simulink model "TranscriticalCO2Cycle"  (R2023b)
settings: Solver=VariableStepAuto  StartTime=0.0  StopTime=10.0  RelTol=1e-3  AbsTol=1e-3
undefined symbols (not defined in the file or in its folder): CO2PropertyTables
libraries: fl_lib x29, SimscapeFluids_lib x7, nesl_utility x1
settings Model: Creator=smemusha  LastModifiedBy=smemusha
settings SolverCC: AutoScaleAbsTol=off  AlgebraicLoopSolver=TrustRegion  MaxZcPerStep=1
settings OptimizationCC: ReuseModelBlockBuffer=off
settings DebuggingCC: UnconnectedInputMsg=warning  UnconnectedOutputMsg=warning  UnconnectedLineMsg=warning  SymbolicDimsDataTypeCodeGenerationDiagnostic=none
settings ModelReferenceCC: EnableRefExpFcnMdlSchedulingChecks=on
settings SFSimCC: CustomCodeUndefinedFunction=UseInterfaceOnly
settings RTWCC: DLArmComputeVersion=19.05
settings SimscapeCC: SimscapeLogType=all  SimscapeLogSimulationStatistics=on  SimscapeLogDataHistory=10000

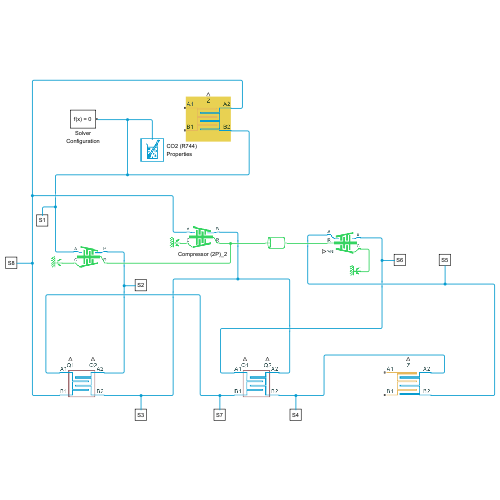
[thumbnail: Simulink's stored preview of the top-level diagram]
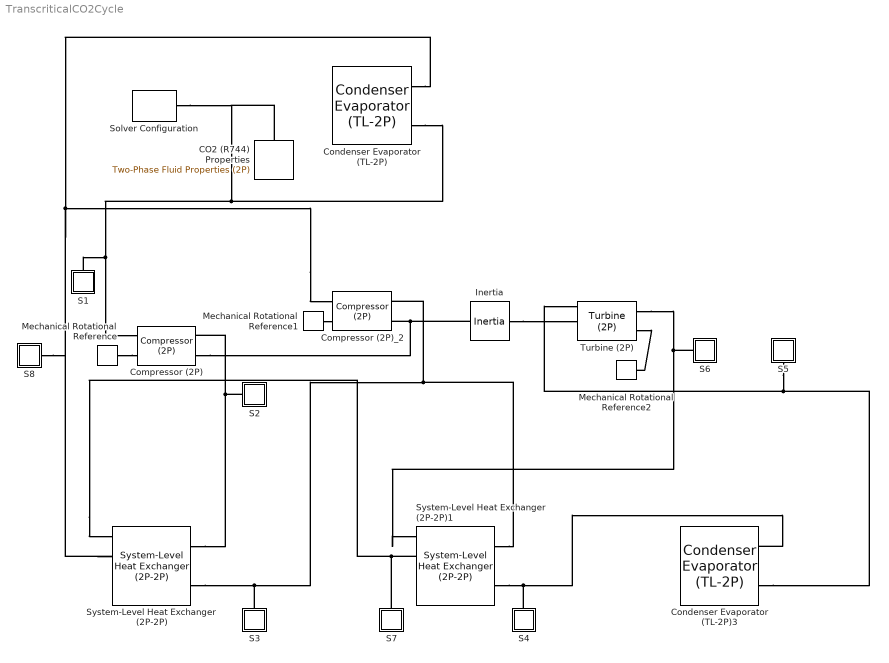
== system TranscriticalCO2Cycle ==
  CO2 (R744) Properties : fl_lib/Two-Phase Fluid/Utilities/Two-Phase Fluid Properties (2P)  u_min=CO2PropertyTables.u_min kJ/kg  u_max=CO2PropertyTables.u_max kJ/kg  p_TLU=CO2PropertyTables.p MPa  p_crit=CO2PropertyTables.p_crit MPa  critical_region=foundation.enum.critical_region.clip  p_crit_fraction=0.12  p_atm=CO2PropertyTables.p(1) MPa  properties_range_check=simscape.enum.assert.action.error  q_rev=0.01 Pa  unorm_liq=CO2PropertyTables.liquid.unorm  v_liq=CO2PropertyTables.liquid.v m^3/kg  s_liq=CO2PropertyTables.liquid.s kJ/kg/K  T_liq=CO2PropertyTables.liquid.T K  nu_liq=CO2PropertyTables.liquid.nu mm^2/s  k_liq=CO2PropertyTables.liquid.k W/(m*K)  Pr_liq=CO2PropertyTables.liquid.Pr  u_sat_liq=CO2PropertyTables.liquid.u_sat kJ/kg  unorm_vap=CO2PropertyTables.vapor.unorm  v_vap=CO2PropertyTables.vapor.v m^3/kg  s_vap=CO2PropertyTables.vapor.s kJ/kg/K  T_vap=CO2PropertyTables.vapor.T K  nu_vap=CO2PropertyTables.vapor.nu m^2/s  k_vap=CO2PropertyTables.vapor.k W/(m*K)  Pr_vap=CO2PropertyTables.vapor.Pr  u_sat_vap=CO2PropertyTables.vapor.u_sat kJ/kg
      settings: InternalSimscapePortConfiguration="{\"Bottom\":[],\"Left\":[],\"Right\":[{\"id\":\"A\",\"label\":\"\",\"type\":\"foundation.two_phase_fluid.two_phase_fluid\"}],\"Top\":[]}"
  Compressor (2P) : SimscapeFluids_lib/Two-Phase Fluid/Fluid Machines/Compressor (2P)  parameterization=fluids.two_phase_fluid.fluid_machines.enum.CompressorParameterization.Analytical  NDes=25000 rpm  piDes=2.2  mdotDes=3 kg/s  efficiencyType=fluids.two_phase_fluid.fluid_machines.enum.EfficiencyType.Analytical  efficiencyValue=0.8  etaMax=0.88  etaMin=0.8  mdotMaxEff=3.5 kg/s  piMaxEff=2.67  omega_TLU=250 .* [50, 71, 87, 100] rpm  beta_TLU=0 : 1 / 5 : 1  pr_TLU=[1.1814, 1.2385, 1.2792, 1.3017, 1.3057, 1.3057; 1.3648, 1.5157, 1.6298, 1.691, 1.7011, 1.7032; 1.587, 1.8357, 2.011, 2.0925, 2.1006, 2.1006; 1.8255, 2.28, 2.4777, 2.5225, 2.5633, 2.5389]  mdot_TLU=[.1503, .1313, .11, .0887, .0668, .0502; .2265, .1999, .1649, .1322, .0992, .0639; .2869, .2545, .216, .1798, .1424, .108; .3275, .2846, .2466, .2285, .209, .1661] kg/s  eta_TLU=[.56, .66, .71, .695, .659, .635; .558, .682, .755, .743, .697, .638; .57, .705, .765, .752, .712, .652; .552, .718, .755, .752, .736, .67]  SMFault=simscape.enum.assert.action.none  a=1.5  b=5  k=0.03  c=3  d=4  cCap=15  dCap=1.0  p_reference=0.101325 MPa  T_reference=373.15 K  mechanical_efficiency=0.9  area_A=0.01 m^2  area_B=0.01 m^2  VaporCheck=simscape.enum.assert.action.warn
      settings: InternalSimscapePortConfiguration="{\"Bottom\":[],\"Left\":[{\"id\":\"A\",\"label\":\"A\",\"type\":\"foundation.two_phase_fluid.two_phase_fluid\"},{\"id\":\"C\",\"label\":\"C\",\"type\":\"foundation.mechanical.rotational.rotational\"}],\"Right\":[{\"id\":\"B\",\"label\":\"B\",\"type\":\"foundation.two_phase_fluid.two_phase_fluid\"},{\"id\":\"R\",\"label\":\"R\",\"type\":\"foundation.mechanical.rotational.rotational\"}],\"Top\":[]}"
  Compressor (2P)_2 : SimscapeFluids_lib/Two-Phase Fluid/Fluid Machines/Compressor (2P)  parameterization=fluids.two_phase_fluid.fluid_machines.enum.CompressorParameterization.Analytical  NDes=25000 rpm  piDes=2.2  mdotDes=0.20 kg/s  efficiencyType=fluids.two_phase_fluid.fluid_machines.enum.EfficiencyType.Analytical  efficiencyValue=0.8  etaMax=0.887  etaMin=0.5  mdotMaxEff=0.19 kg/s  piMaxEff=2.1  omega_TLU=250 .* [50, 71, 87, 100] rpm  beta_TLU=0 : 1 / 5 : 1  pr_TLU=[1.1814, 1.2385, 1.2792, 1.3017, 1.3057, 1.3057; 1.3648, 1.5157, 1.6298, 1.691, 1.7011, 1.7032; 1.587, 1.8357, 2.011, 2.0925, 2.1006, 2.1006; 1.8255, 2.28, 2.4777, 2.5225, 2.5633, 2.5389]  mdot_TLU=[.1503, .1313, .11, .0887, .0668, .0502; .2265, .1999, .1649, .1322, .0992, .0639; .2869, .2545, .216, .1798, .1424, .108; .3275, .2846, .2466, .2285, .209, .1661] kg/s  eta_TLU=[.56, .66, .71, .695, .659, .635; .558, .682, .755, .743, .697, .638; .57, .705, .765, .752, .712, .652; .552, .718, .755, .752, .736, .67]  SMFault=simscape.enum.assert.action.none  a=1.5  b=5  k=0.03  c=3  d=4  cCap=15  dCap=1.0  p_reference=0.101325 MPa  T_reference=373.15 K  mechanical_efficiency=0.9  area_A=0.01 m^2  area_B=0.01 m^2  VaporCheck=simscape.enum.assert.action.warn
      settings: InternalSimscapePortConfiguration="{\"Bottom\":[],\"Left\":[{\"id\":\"A\",\"label\":\"A\",\"type\":\"foundation.two_phase_fluid.two_phase_fluid\"},{\"id\":\"C\",\"label\":\"C\",\"type\":\"foundation.mechanical.rotational.rotational\"}],\"Right\":[{\"id\":\"B\",\"label\":\"B\",\"type\":\"foundation.two_phase_fluid.two_phase_fluid\"},{\"id\":\"R\",\"label\":\"R\",\"type\":\"foundation.mechanical.rotational.rotational\"}],\"Top\":[]}"
  Condenser Evaporator (TL-2P) : SimscapeFluids_lib/Fluid Network Interfaces/Heat Exchangers/Condenser Evaporator (TL-2P)  flow_arrangement=fluids.interfaces.heat_exchangers.enum.FlowArrangementTL2P.Cross  cross_flow_arrangement=fluids.interfaces.heat_exchangers.enum.CrossFlowArrangementTL2P.UnmixedUnmixed  R_wall=0 K/kW  area_A1=0.01 m^2  area_B1=0.01 m^2  area_A2=0.01 m^2  area_B2=0.01 m^2  flow_geometry_TL=fluids.interfaces.heat_exchangers.enum.FlowGeometryTL.InsideTubes  tube_num_TL=25  tube_length_TL=1 m  tube_cross_section_TL=fluids.interfaces.heat_exchangers.enum.TubeCrossSection.Circular  tube_diameter_TL=0.05 m  tube_width_TL=0.05 m  tube_height_TL=0.05 m  tube_inner_diameter_TL=0.05 m  tube_outer_diameter_TL=0.1 m  tube_flow_area_TL=0.002 m^2  tube_wetted_perimeter_TL=0.15 m  tube_heat_perimeter_TL=0.15 m  tube_pressure_loss_spec_TL=fluids.interfaces.heat_exchangers.enum.TubePressureLossSpec.Haaland  tube_loss_coeff_TL=10  tube_local_pressure_loss_spec_TL=fluids.thermal_liquid.pipes_fittings.enum.LocalLossSpec.AggregateLength  tube_length_add_TL=0.1 m  tube_local_loss_coefficient_TL=0.1  tube_roughness_pressure_TL=15e-6 m  tube_Re_lam_pressure_TL=2000  tube_Re_tur_pressure_TL=4000  tube_shape_factor_generic_TL=64  tube_heat_coeff_spec_TL=fluids.interfaces.heat_exchangers.enum.TubeHeatCoeffSpec.Gneilinski  tube_colburn_coeff_TL=[.023, .8, .33]  tube_roughness_heat_TL=15e-6 m  tube_Re_lam_heat_TL=2000  tube_Re_tur_heat_TL=4000  tube_Nu_lam_generic_TL=3.66  bank_arrangement_TL=fluids.interfaces.heat_exchangers.enum.BankArrangement.Inline  bank_num_rows_TL=5  bank_tubes_per_row_TL=5  bank_width_TL=1 m  bank_tube_diameter_TL=0.05 m  bank_longitudinal_pitch_TL=0.15 m  bank_transverse_pitch_TL=0.15 m  bank_pressure_loss_spec_TL=fluids.interfaces.heat_exchangers.enum.BankPressureLossSpec.Martin  bank_euler_TL=10  bank_heat_coeff_spec_TL=fluids.interfaces.heat_exchangers.enum.BankHeatCoeffSpec.Martin  bank_colburn_coeff_TL=[.27, .63, .36]  generic_flow_area_TL=0.01 m^2  generic_heat_area_TL=2 m^2  generic_volume_TL=0.05 m^3  generic_loss_coeff_TL=10  generic_colburn_coeff_TL=[.023, .8, .33]  fouling_factor_TL=0.1 K*m^2/kW  fin_area_TL=0 m^2  fin_efficiency_TL=0.5  p_init_TL=7.5 MPa  T_init_TL=305 K  tube_num_2P=25  tube_length_2P=1 m  tube_cross_section_2P=fluids.interfaces.heat_exchangers.enum.TubeCrossSection.Circular  tube_diameter_2P=0.05 m  tube_width_2P=0.05 m  tube_height_2P=0.05 m  tube_inner_diameter_2P=0.05 m  tube_outer_diameter_2P=0.1 m  tube_flow_area_2P=0.002 m^2  tube_wetted_perimeter_2P=0.15 m  tube_heat_perimeter_2P=0.15 m  tube_pressure_loss_spec_2P=fluids.interfaces.heat_exchangers.enum.TubePressureLossSpec2P.Haaland  tube_loss_coeff_2P=10  tube_local_pressure_loss_spec_2P=fluids.two_phase_fluid.pipes_fittings.enum.LocalLossSpec.AggregateLength  tube_length_add_2P=0.1 m  tube_local_loss_coefficient_2P=0.1  tube_roughness_pressure_2P=15e-6 m  tube_Re_lam_pressure_2P=2000  tube_Re_tur_pressure_2P=4000  tube_shape_factor_generic_2P=64  tube_heat_coeff_spec_2P=fluids.interfaces.heat_exchangers.enum.TubeHeatCoeffSpec2P.GneilinskiCavalliniZecchin  tube_colburn_coeff_liq_2P=[.023, .8, .33]  tube_colburn_coeff_mix_2P=[.05, .8, .33]  tube_colburn_coeff_vap_2P=[.023, .8, .33]  tube_roughness_heat_2P=15e-6 m  tube_Re_lam_heat_2P=2000  tube_Re_tur_heat_2P=4000  tube_Nu_lam_generic_2P=3.66  fouling_factor_2P=0.1 K*m^2/kW  fin_area_2P=0 m^2  fin_efficiency_2P=0.5  energy_spec_2P=foundation.enum.energy_spec.temperature  p_init_2P=0.101325 MPa  T_init_2P=293.15 K  x_init_2P=0.5  alpha_init_2P=0.5  h_init_2P=1500 kJ/kg  u_init_2P=1500 kJ/kg
      settings: InternalSimscapePortConfiguration="{\"Bottom\":[],\"Left\":[{\"id\":\"A1\",\"label\":\"A1\",\"type\":\"foundation.thermal_liquid.thermal_liquid\"},{\"id\":\"B1\",\"label\":\"B1\",\"type\":\"foundation.thermal_liquid.thermal_liquid\"}],\"Right\":[{\"id\":\"A2\",\"label\":\"A2\",\"type\":\"foundation.two_phase_fluid.two_phase_fluid\"},{\"id\":\"B2\",\"label\":\"B2\",\"type\":\"foundation.two_phase_fluid.two_phase_fluid\"}],\"Top\":[{\"id\":\"Z\",\"label\":\"Z\",\"type\":\"output\"}]}"
  Condenser Evaporator (TL-2P)3 : SimscapeFluids_lib/Fluid Network Interfaces/Heat Exchangers/Condenser Evaporator (TL-2P)  flow_arrangement=fluids.interfaces.heat_exchangers.enum.FlowArrangementTL2P.Cross  cross_flow_arrangement=fluids.interfaces.heat_exchangers.enum.CrossFlowArrangementTL2P.UnmixedUnmixed  R_wall=0 K/kW  area_A1=0.01 m^2  area_B1=0.01 m^2  area_A2=0.01 m^2  area_B2=0.01 m^2  flow_geometry_TL=fluids.interfaces.heat_exchangers.enum.FlowGeometryTL.InsideTubes  tube_num_TL=25  tube_length_TL=1 m  tube_cross_section_TL=fluids.interfaces.heat_exchangers.enum.TubeCrossSection.Circular  tube_diameter_TL=0.05 m  tube_width_TL=0.05 m  tube_height_TL=0.05 m  tube_inner_diameter_TL=0.05 m  tube_outer_diameter_TL=0.1 m  tube_flow_area_TL=0.002 m^2  tube_wetted_perimeter_TL=0.15 m  tube_heat_perimeter_TL=0.15 m  tube_pressure_loss_spec_TL=fluids.interfaces.heat_exchangers.enum.TubePressureLossSpec.Haaland  tube_loss_coeff_TL=10  tube_local_pressure_loss_spec_TL=fluids.thermal_liquid.pipes_fittings.enum.LocalLossSpec.AggregateLength  tube_length_add_TL=0.1 m  tube_local_loss_coefficient_TL=0.1  tube_roughness_pressure_TL=15e-6 m  tube_Re_lam_pressure_TL=2000  tube_Re_tur_pressure_TL=4000  tube_shape_factor_generic_TL=64  tube_heat_coeff_spec_TL=fluids.interfaces.heat_exchangers.enum.TubeHeatCoeffSpec.Gneilinski  tube_colburn_coeff_TL=[.023, .8, .33]  tube_roughness_heat_TL=15e-6 m  tube_Re_lam_heat_TL=2000  tube_Re_tur_heat_TL=4000  tube_Nu_lam_generic_TL=3.66  bank_arrangement_TL=fluids.interfaces.heat_exchangers.enum.BankArrangement.Inline  bank_num_rows_TL=5  bank_tubes_per_row_TL=5  bank_width_TL=1 m  bank_tube_diameter_TL=0.05 m  bank_longitudinal_pitch_TL=0.15 m  bank_transverse_pitch_TL=0.15 m  bank_pressure_loss_spec_TL=fluids.interfaces.heat_exchangers.enum.BankPressureLossSpec.Martin  bank_euler_TL=10  bank_heat_coeff_spec_TL=fluids.interfaces.heat_exchangers.enum.BankHeatCoeffSpec.Martin  bank_colburn_coeff_TL=[.27, .63, .36]  generic_flow_area_TL=0.01 m^2  generic_heat_area_TL=2 m^2  generic_volume_TL=0.05 m^3  generic_loss_coeff_TL=10  generic_colburn_coeff_TL=[.023, .8, .33]  fouling_factor_TL=0.1 K*m^2/kW  fin_area_TL=0 m^2  fin_efficiency_TL=0.5  p_init_TL=0.101325 MPa  T_init_TL=293.15 K  tube_num_2P=25  tube_length_2P=1 m  tube_cross_section_2P=fluids.interfaces.heat_exchangers.enum.TubeCrossSection.Circular  tube_diameter_2P=0.05 m  tube_width_2P=0.05 m  tube_height_2P=0.05 m  tube_inner_diameter_2P=0.05 m  tube_outer_diameter_2P=0.1 m  tube_flow_area_2P=0.002 m^2  tube_wetted_perimeter_2P=0.15 m  tube_heat_perimeter_2P=0.15 m  tube_pressure_loss_spec_2P=fluids.interfaces.heat_exchangers.enum.TubePressureLossSpec2P.Haaland  tube_loss_coeff_2P=10  tube_local_pressure_loss_spec_2P=fluids.two_phase_fluid.pipes_fittings.enum.LocalLossSpec.AggregateLength  tube_length_add_2P=0.1 m  tube_local_loss_coefficient_2P=0.1  tube_roughness_pressure_2P=15e-6 m  tube_Re_lam_pressure_2P=2000  tube_Re_tur_pressure_2P=4000  tube_shape_factor_generic_2P=64  tube_heat_coeff_spec_2P=fluids.interfaces.heat_exchangers.enum.TubeHeatCoeffSpec2P.GneilinskiCavalliniZecchin  tube_colburn_coeff_liq_2P=[.023, .8, .33]  tube_colburn_coeff_mix_2P=[.05, .8, .33]  tube_colburn_coeff_vap_2P=[.023, .8, .33]  tube_roughness_heat_2P=15e-6 m  tube_Re_lam_heat_2P=2000  tube_Re_tur_heat_2P=4000  tube_Nu_lam_generic_2P=3.66  fouling_factor_2P=0.1 K*m^2/kW  fin_area_2P=0 m^2  fin_efficiency_2P=0.5  energy_spec_2P=foundation.enum.energy_spec.temperature  p_init_2P=0.101325 MPa  T_init_2P=293.15 K  x_init_2P=0.5  alpha_init_2P=0.5  h_init_2P=1500 kJ/kg  u_init_2P=1500 kJ/kg
      settings: InternalSimscapePortConfiguration="{\"Bottom\":[],\"Left\":[{\"id\":\"A1\",\"label\":\"A1\",\"type\":\"foundation.thermal_liquid.thermal_liquid\"},{\"id\":\"B1\",\"label\":\"B1\",\"type\":\"foundation.thermal_liquid.thermal_liquid\"}],\"Right\":[{\"id\":\"A2\",\"label\":\"A2\",\"type\":\"foundation.two_phase_fluid.two_phase_fluid\"},{\"id\":\"B2\",\"label\":\"B2\",\"type\":\"foundation.two_phase_fluid.two_phase_fluid\"}],\"Top\":[{\"id\":\"Z\",\"label\":\"Z\",\"type\":\"output\"}]}"
  Inertia : fl_lib/Mechanical/Rotational Elements/Inertia  inertia=shaft_inertia kg*m^2  num_ports=foundation.enum.numPorts2.two  w_specify=on  w_priority=High  w=10000 rpm  w_nominal_specify=off  w_nominal_unit=rad/s  w_nominal_value=1  t_specify=off  t_priority=None  t=0 N*m  t_nominal_specify=off  t_nominal_unit=N*m  t_nominal_value=1
      settings: InternalSimscapePortConfiguration="{\"Bottom\":[],\"Left\":[{\"id\":\"I\",\"label\":\"\",\"type\":\"foundation.mechanical.rotational.rotational\"}],\"Right\":[{\"id\":\"J\",\"label\":\"\",\"type\":\"foundation.mechanical.rotational.rotational\"}],\"Top\":[]}"
  Mechanical Rotational Reference : fl_lib/Mechanical/Rotational Elements/Mechanical Rotational Reference
  Mechanical Rotational Reference1 : fl_lib/Mechanical/Rotational Elements/Mechanical Rotational Reference
  Mechanical Rotational Reference2 : fl_lib/Mechanical/Rotational Elements/Mechanical Rotational Reference
  S1 : Subsystem
      mask Display: disp(get_param(gcb, 'Name'))
  S2 : Subsystem
      settings: PortSchema="{\"entries\":[{\"content\":{\"sides\":[{\"content\":{},\"type\":\"ConnectorPlacement.EquallySpacedRectSide\",\"uuid\":\"af0e4199-d47a-4ec0-94eb-7962f8049a35\"},{\"content\":{\"side\":\"RIGHT\"},\"type\":\"ConnectorPlacement.EquallySpacedRectSide\",\"uuid\":\"e53baceb-841d-4d18-830d-da2777b33e2d\"},{\"content\":{\"connectorIds\":[\"LConn1\"],\"side\":\"TOP\"},\"type\":\"ConnectorPlacement.EquallySpacedRectSide\",\"uuid\":\"c9dd45b9-7dec-4baa-8c3e-b872dab8c4af\"}]},\"type\":\"ConnectorPlacement.EquallySpacedConnector\",\"uuid\":\"6eb31624-81b7-422d-8922-37e9cf91a1f7\"}],\"packageUris\":[\"http://schema.mathworks.com/mf0/Connector/R2020b\"],\"version\":\"1.0\"}"
      mask Display: disp(get_param(gcb, 'Name'))
  S3 : Subsystem
      mask Display: disp(get_param(gcb, 'Name'))
  S4 : Subsystem
      mask Display: disp(get_param(gcb, 'Name'))
  S5 : Subsystem
      mask Display: disp(get_param(gcb, 'Name'))
  S6 : Subsystem
      settings: PortSchema="{\"entries\":[{\"content\":{\"sides\":[{\"content\":{},\"type\":\"ConnectorPlacement.EquallySpacedRectSide\",\"uuid\":\"af0e4199-d47a-4ec0-94eb-7962f8049a35\"},{\"content\":{\"side\":\"RIGHT\"},\"type\":\"ConnectorPlacement.EquallySpacedRectSide\",\"uuid\":\"e53baceb-841d-4d18-830d-da2777b33e2d\"},{\"content\":{\"connectorIds\":[\"LConn1\"],\"side\":\"TOP\"},\"type\":\"ConnectorPlacement.EquallySpacedRectSide\",\"uuid\":\"c9dd45b9-7dec-4baa-8c3e-b872dab8c4af\"}]},\"type\":\"ConnectorPlacement.EquallySpacedConnector\",\"uuid\":\"6eb31624-81b7-422d-8922-37e9cf91a1f7\"}],\"packageUris\":[\"http://schema.mathworks.com/mf0/Connector/R2020b\"],\"version\":\"1.0\"}"
      mask Display: disp(get_param(gcb, 'Name'))
  S7 : Subsystem
      mask Display: disp(get_param(gcb, 'Name'))
  S8 : Subsystem
      settings: PortSchema="{\"entries\":[{\"content\":{\"sides\":[{\"content\":{},\"type\":\"ConnectorPlacement.EquallySpacedRectSide\",\"uuid\":\"af0e4199-d47a-4ec0-94eb-7962f8049a35\"},{\"content\":{\"side\":\"RIGHT\"},\"type\":\"ConnectorPlacement.EquallySpacedRectSide\",\"uuid\":\"e53baceb-841d-4d18-830d-da2777b33e2d\"},{\"content\":{\"side\":\"TOP\"},\"type\":\"ConnectorPlacement.EquallySpacedRectSide\",\"uuid\":\"c9dd45b9-7dec-4baa-8c3e-b872dab8c4af\"},{\"content\":{\"connectorIds\":[\"RConn1\"],\"side\":\"BOTTOM\"},\"type\":\"ConnectorPlacement.EquallySpacedRectSide\",\"uuid\":\"10f1a485-95f0-4282-b277-18e46c743bab\"}]},\"type\":\"ConnectorPlacement.EquallySpacedConnector\",\"uuid\":\"6eb31624-81b7-422d-8922-37e9cf91a1f7\"}],\"packageUris\":[\"http://schema.mathworks.com/mf0/Connector/R2020b\"],\"version\":\"1.0\"}"
      mask Display: disp(get_param(gcb, 'Name'))
  Solver Configuration : nesl_utility/Solver Configuration  PhysicalDomain=network_engine_domain  SubClassName=solver  LeftPortType=input  RightPortType=generic  Tones=[]  Harmonics=[]  SimulateNoise=off  Profile=off  UseLocalSampling=off  EnableSwitchedLinearOptims=on  FrequencyDomain=off  UseCCode=off  RelTol=0.001  AbsTol=1e-06  MinStep=1e-09  ToWorkspace=off  RevertToSquareIcSolve=off  NumHomotopyIterations=100  PhasorMode=off  PhasorModeNumHarmonics=1  ConsistencySolver=NEWTON_XTOL_AFTER_FTOL  IndexReductionMethod=DerivativeReplacement  DoDC=off  ResidualTolerance=1e-09  ConsistencyTolSource=GLOBAL  ConsistencyAbsTol=0.001  ConsistencyRelTol=0.001  ConsistencyTolFactor=0.001  UseLocalSolver=off  LocalSolverChoice=NE_BACKWARD_EULER_ADVANCER  ResolveIndetEquations=on  FunctionEvalNumThread=1  LocalSolverSampleTime=0.001  DoFixedCost=off  MaxNonlinIter=3  MaxModeIter=2  ComputeImpulses=off  ImpulseIterations=2  LinearAlgebra=auto  LinearAlgebraNumThread=0  EquationFormulation=NE_TIME_EF  DelaysMemoryBudget=1024  AutomaticFiltering=on  FilteringTimeConstant=0.001  PartitionStorageMethod=AS_NEEDED  PartitionMemoryBudget=1024  PartitionMethod=ROBUST  MultibodyUseLocalSolver=off  MultibodyLocalSolverChoice=ODE1  MultibodyLocalSolverSampleTime=0.001
  System-Level Heat Exchanger (2P-2P) : SimscapeFluids_lib/Fluid Network Interfaces/Heat Exchangers/System-Level Heat Exchanger (2P-2P)  flow_arrangement=fluids.interfaces.heat_exchangers.enum.SystemLevelFlowArrangement2P2P.Counter  wall_thermal_mass=false  mass_wall=1 kg  cp_wall=490 J/(K*kg)  nominal_init_wall=true  T_wall_init=293.15 K  area_A1=0.01 m^2  area_B1=0.01 m^2  area_A2=0.01 m^2  area_B2=0.01 m^2  operating_condition_2P1=fluids.interfaces.heat_exchangers.enum.SystemLevelOperatingCondition2P2P.Cooling  mdot_nominal_2P1=0.001 kg/s  delta_p_nominal_2P1=0.01 MPa  pressure_spec_2P1=fluids.interfaces.heat_exchangers.enum.SystemLevelPressureSpec2P.InletPressure  p_in_nominal_2P1=1 MPa  T_sat_nominal_2P1=313.15 K  inlet_spec_2P1=fluids.interfaces.heat_exchangers.enum.SystemLevelInletSpec2P.Enthalpy  T_in_nominal_2P1=333.15 K  h_in_nominal_2P1=440 kJ/kg  x_in_nominal_2P1=1  capacity_spec_2P1=fluids.interfaces.heat_exchangers.enum.SystemLevelCapacitySpec.HeatTransfer  Q_nominal=0.1 kW  outlet_spec_cool_2P1=fluids.interfaces.heat_exchangers.enum.SystemLevelOutletSpecCondenser2P.Enthalpy  outlet_spec_heat_2P1=fluids.interfaces.heat_exchangers.enum.SystemLevelOutletSpecEvaporator2P.Enthalpy  delta_T_sub_nominal_2P1=5 deltaK  delta_T_sup_nominal_2P1=5 deltaK  h_out_nominal_2P1=250 kJ/kg  x_out_nominal_2P1=0  volume_2P1=0.001 m^3  nominal_init_2P1=true  energy_spec_2P1=foundation.enum.energy_spec.enthalpy  p_init_2P1=0.101325 MPa  T_init_2P1=293.15 K  x_init_2P1=0.5  alpha_init_2P1=0.5  h_init_2P1=1500 kJ/kg  u_init_2P1=1500 kJ/kg  mdot_nominal_2P2=0.001 kg/s  delta_p_nominal_2P2=0.01 MPa  pressure_spec_2P2=fluids.interfaces.heat_exchangers.enum.SystemLevelPressureSpec2P.InletPressure  p_in_nominal_2P2=0.1 MPa  T_sat_nominal_2P2=243.15 K  inlet_spec_2P2=fluids.interfaces.heat_exchangers.enum.SystemLevelInletSpec2P.Enthalpy  T_in_nominal_2P2=237.15 K  h_in_nominal_2P2=230 kJ/kg  x_in_nominal_2P2=0.1  volume_2P2=0.001 m^3  nominal_init_2P2=true  energy_spec_2P2=foundation.enum.energy_spec.enthalpy  p_init_2P2=0.101325 MPa  T_init_2P2=293.15 K  x_init_2P2=0.5  alpha_init_2P2=0.5  h_init_2P2=1500 kJ/kg  u_init_2P2=1500 kJ/kg  a_liq_2P1=0.023  a_mix_2P1=0.005  a_vap_2P1=0.023  b_2P1=0.8  c_2P1=0.33  a_liq_2P2=0.023  a_mix_2P2=0.005  a_vap_2P2=0.023  b_2P2=0.8  c_2P2=0.33
      settings: InternalSimscapePortConfiguration="{\"Bottom\":[],\"Left\":[{\"id\":\"A1\",\"label\":\"A1\",\"type\":\"foundation.two_phase_fluid.two_phase_fluid\"},{\"id\":\"B1\",\"label\":\"B1\",\"type\":\"foundation.two_phase_fluid.two_phase_fluid\"}],\"Right\":[{\"id\":\"A2\",\"label\":\"A2\",\"type\":\"foundation.two_phase_fluid.two_phase_fluid\"},{\"id\":\"B2\",\"label\":\"B2\",\"type\":\"foundation.two_phase_fluid.two_phase_fluid\"}],\"Top\":[{\"id\":\"Q1\",\"label\":\"Q1\",\"type\":\"output\"},{\"id\":\"Q2\",\"label\":\"Q2\",\"type\":\"output\"}]}"
  System-Level Heat Exchanger (2P-2P)1 : SimscapeFluids_lib/Fluid Network Interfaces/Heat Exchangers/System-Level Heat Exchanger (2P-2P)  flow_arrangement=fluids.interfaces.heat_exchangers.enum.SystemLevelFlowArrangement2P2P.Counter  wall_thermal_mass=false  mass_wall=1 kg  cp_wall=490 J/(K*kg)  nominal_init_wall=true  T_wall_init=293.15 K  area_A1=0.01 m^2  area_B1=0.01 m^2  area_A2=0.01 m^2  area_B2=0.01 m^2  operating_condition_2P1=fluids.interfaces.heat_exchangers.enum.SystemLevelOperatingCondition2P2P.Cooling  mdot_nominal_2P1=0.001 kg/s  delta_p_nominal_2P1=0.01 MPa  pressure_spec_2P1=fluids.interfaces.heat_exchangers.enum.SystemLevelPressureSpec2P.InletPressure  p_in_nominal_2P1=1 MPa  T_sat_nominal_2P1=313.15 K  inlet_spec_2P1=fluids.interfaces.heat_exchangers.enum.SystemLevelInletSpec2P.Enthalpy  T_in_nominal_2P1=333.15 K  h_in_nominal_2P1=440 kJ/kg  x_in_nominal_2P1=1  capacity_spec_2P1=fluids.interfaces.heat_exchangers.enum.SystemLevelCapacitySpec.HeatTransfer  Q_nominal=0.1 kW  outlet_spec_cool_2P1=fluids.interfaces.heat_exchangers.enum.SystemLevelOutletSpecCondenser2P.Enthalpy  outlet_spec_heat_2P1=fluids.interfaces.heat_exchangers.enum.SystemLevelOutletSpecEvaporator2P.Enthalpy  delta_T_sub_nominal_2P1=5 deltaK  delta_T_sup_nominal_2P1=5 deltaK  h_out_nominal_2P1=250 kJ/kg  x_out_nominal_2P1=0  volume_2P1=0.001 m^3  nominal_init_2P1=true  energy_spec_2P1=foundation.enum.energy_spec.enthalpy  p_init_2P1=0.101325 MPa  T_init_2P1=293.15 K  x_init_2P1=0.5  alpha_init_2P1=0.5  h_init_2P1=1500 kJ/kg  u_init_2P1=1500 kJ/kg  mdot_nominal_2P2=0.001 kg/s  delta_p_nominal_2P2=0.01 MPa  pressure_spec_2P2=fluids.interfaces.heat_exchangers.enum.SystemLevelPressureSpec2P.InletPressure  p_in_nominal_2P2=0.1 MPa  T_sat_nominal_2P2=243.15 K  inlet_spec_2P2=fluids.interfaces.heat_exchangers.enum.SystemLevelInletSpec2P.Enthalpy  T_in_nominal_2P2=237.15 K  h_in_nominal_2P2=230 kJ/kg  x_in_nominal_2P2=0.1  volume_2P2=0.001 m^3  nominal_init_2P2=true  energy_spec_2P2=foundation.enum.energy_spec.enthalpy  p_init_2P2=0.101325 MPa  T_init_2P2=293.15 K  x_init_2P2=0.5  alpha_init_2P2=0.5  h_init_2P2=1500 kJ/kg  u_init_2P2=1500 kJ/kg  a_liq_2P1=0.023  a_mix_2P1=0.005  a_vap_2P1=0.023  b_2P1=0.8  c_2P1=0.33  a_liq_2P2=0.023  a_mix_2P2=0.005  a_vap_2P2=0.023  b_2P2=0.8  c_2P2=0.33
      settings: InternalSimscapePortConfiguration="{\"Bottom\":[],\"Left\":[{\"id\":\"A1\",\"label\":\"A1\",\"type\":\"foundation.two_phase_fluid.two_phase_fluid\"},{\"id\":\"B1\",\"label\":\"B1\",\"type\":\"foundation.two_phase_fluid.two_phase_fluid\"}],\"Right\":[{\"id\":\"A2\",\"label\":\"A2\",\"type\":\"foundation.two_phase_fluid.two_phase_fluid\"},{\"id\":\"B2\",\"label\":\"B2\",\"type\":\"foundation.two_phase_fluid.two_phase_fluid\"}],\"Top\":[{\"id\":\"Q1\",\"label\":\"Q1\",\"type\":\"output\"},{\"id\":\"Q2\",\"label\":\"Q2\",\"type\":\"output\"}]}"
  Turbine (2P) : SimscapeFluids_lib/Two-Phase Fluid/Fluid Machines/Turbine (2P)  parameterization=fluids.two_phase_fluid.fluid_machines.enum.TurbineParameterization.Analytical  omega_TLU_2=250 .* [50, 60, 70, 80, 90, 100, 110] rpm  variable_nozzle=true  min_nozzle_opening=1e-3  max_nozzle_opening=1  pr_nom=2.67  mdot_nom=3 kg/s  pr_mdot_TLU=[1.251, 1.345, 1.442, 1.521, 1.596, 1.692, 1.849, 1.972, 2.1, 2.173, 2.259, 2.3424]  mdot_TLU=0.01 .* [39.439, 43.01, 45.556, 46.801, 47.792, 48.388, 48.634, 48.67, 48.689, 48.747, 48.825, 48.912] kg/s  pr_mdot_TLU_2=[1.217, 1.285, 1.323, 1.363, 1.402, 1.427, 1.495, 1.545, 1.6, 1.687, 1.747, 1.8074; 1.231, 1.302, 1.356, 1.404, 1.443, 1.473, 1.525, 1.577, 1.635, 1.709, 1.782, 1.845; 1.242, 1.328, 1.388, 1.437, 1.528, 1.617, 1.704, 1.811, 1.915, 1.979, 2.053, 2.1226; 1.244, 1.339, 1.417, 1.465, 1.528, 1.584, 1.692, 1.787, 1.899, 2, 2.075, 2.1492; 1.245, 1.34, 1.425, 1.492, 1.546, 1.684, 1.748, 1.882, 1.987, 2.084, 2.167, 2.2458; 1.251, 1.345, 1.442, 1.521, 1.596, 1.692, 1.849, 1.972, 2.1, 2.173, 2.259, 2.3424; 1.248, 1.348, 1.447, 1.516, 1.581, 1.651, 1.749, 1.839, 1.93, 2.024, 2.154, 2.242]  mdot_TLU_2=0.01 .* [40.403, 44.417, 46.653, 47.966, 48.97, 49.544, 50.001, 50.081, 50.086, 50.095, 50.09, 50.0922; 40.044, 43.754, 46.125, 47.626, 48.513, 49.105, 49.481, 49.58, 49.597, 49.624, 49.638, 49.633; 39.941, 43.795, 46.017, 47.335, 48.795, 49.199, 49.279, 49.27, 49.248, 49.23, 49.255, 49.2428; 39.896, 43.512, 45.914, 47.061, 48.011, 48.558, 48.943, 49.042, 49.069, 49.01, 49.046, 49.0266; 39.524, 42.934, 45.686, 46.743, 47.715, 48.67, 48.777, 48.836, 48.876, 48.836, 48.845, 48.8184; 39.439, 43.01, 45.556, 46.801, 47.792, 48.388, 48.634, 48.67, 48.639, 48.647, 48.625, 48.5912; 39.502, 42.849, 45.336, 46.385, 47.312, 47.877, 48.222, 48.397, 48.459, 48.482, 48.455, 48.414] kg/s  efficiency_constant=0.9  pr_eta_TLU=[1.252, 1.328, 1.425, 1.544, 1.642, 1.757, 1.873, 2.005, 2.1, 2.204, 2.248, 2.28]  eta_TLU=[.559, .61, .673, .741, .788, .835, .869, .895, .908, .899, .854, .751]  pr_eta_TLU_2=[1.224, 1.246, 1.292, 1.387, 1.457, 1.534, 1.61, 1.686, 1.743, 1.79, 1.871, 1.914; 1.237, 1.25, 1.28, 1.369, 1.459, 1.553, 1.629, 1.716, 1.799, 1.846, 1.927, 1.97; 1.241, 1.255, 1.283, 1.326, 1.401, 1.509, 1.591, 1.704, 1.806, 1.913, 1.994, 2.037; 1.25, 1.265, 1.308, 1.364, 1.456, 1.532, 1.637, 1.739, 1.851, 1.934, 2.042, 2.085; 1.281, 1.314, 1.371, 1.425, 1.498, 1.574, 1.647, 1.749, 1.878, 1.979, 2.091, 2.18; 1.252, 1.328, 1.425, 1.544, 1.642, 1.757, 1.873, 2.005, 2.1, 2.204, 2.248, 2.28; 1.382, 1.43, 1.495, 1.586, 1.688, 1.791, 1.887, 1.99, 2.079, 2.158, 2.249, 2.36]  eta_TLU_2=[.72, .754, .759, .739, .714, .679, .643, .603, .554, .524, .494, .48; .716, .757, .794, .819, .812, .788, .761, .728, .692, .662, .632, .618; .629, .691, .775, .831, .858, .869, .859, .842, .816, .782, .752, .738; .594, .668, .757, .804, .857, .883, .892, .893, .884, .865, .835, .821; .664, .72, .779, .823, .858, .883, .897, .905, .904, .896, .883, .868; .559, .61, .673, .741, .788, .835, .869, .895, .908, .899, .854, .751; .718, .785, .824, .855, .882, .9, .908, .906, .884, .857, .804, .701]  p_reference=0.101325 MPa  T_reference=373.15 K  mechanical_efficiency=0.9  area_A=0.01 m^2  area_B=0.01 m^2  vapor_check=simscape.enum.assert.action.warn
      settings: InternalSimscapePortConfiguration="{\"Bottom\":[],\"Left\":[{\"id\":\"A\",\"label\":\"A\",\"type\":\"foundation.two_phase_fluid.two_phase_fluid\"},{\"id\":\"R\",\"label\":\"R\",\"type\":\"foundation.mechanical.rotational.rotational\"},{\"id\":\"VN\",\"label\":\"VN\",\"type\":\"input\"}],\"Right\":[{\"id\":\"B\",\"label\":\"B\",\"type\":\"foundation.two_phase_fluid.two_phase_fluid\"},{\"id\":\"C\",\"label\":\"C\",\"type\":\"foundation.mechanical.rotational.rotational\"}],\"Top\":[]}"
  connections:
  Condenser Evaporator (TL-2P)/RConn2 -- CO2 (R744) Properties/RConn1 -- Solver Configuration/RConn1 -- S1/LConn1 -- Compressor (2P)/LConn1
  System-Level Heat Exchanger (2P-2P)/RConn1 -- Compressor (2P)/RConn1 -- S2/LConn1
  System-Level Heat Exchanger (2P-2P)/RConn2 -- S3/LConn1 -- System-Level Heat Exchanger (2P-2P)1/RConn1 -- Compressor (2P)_2/RConn1
  System-Level Heat Exchanger (2P-2P)1/RConn2 -- S4/LConn1 -- Condenser Evaporator (TL-2P)3/RConn1
  Condenser Evaporator (TL-2P)3/RConn2 -- S5/RConn1 -- Turbine (2P)/LConn1
  Turbine (2P)/RConn1 -- S6/LConn1 -- System-Level Heat Exchanger (2P-2P)1/LConn1
  System-Level Heat Exchanger (2P-2P)1/LConn2 -- S7/LConn1 -- System-Level Heat Exchanger (2P-2P)/LConn1
  System-Level Heat Exchanger (2P-2P)/LConn2 -- S8/RConn1 -- Condenser Evaporator (TL-2P)/RConn1 -- Compressor (2P)_2/LConn1
  Mechanical Rotational Reference/LConn1 -- Compressor (2P)/LConn2
  Mechanical Rotational Reference1/LConn1 -- Compressor (2P)_2/LConn2
  Turbine (2P)/RConn2 -- Mechanical Rotational Reference2/LConn1
  Inertia/LConn1 -- Compressor (2P)/RConn2 -- Compressor (2P)_2/RConn2
  Inertia/RConn1 -- Turbine (2P)/LConn2

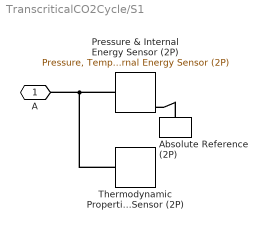
== system TranscriticalCO2Cycle/S1 ==
  Absolute Reference (2P) : fl_lib/Two-Phase Fluid/Elements/Absolute Reference (2P)
  Pressure & Internal Energy Sensor (2P) : fl_lib/Two-Phase Fluid/Sensors/Pressure, Temperature & Internal Energy Sensor (2P)  reference=foundation.enum.MeasurementReference.difference  pressure=true  pressure_spec=foundation.enum.PressureMeasementSpec.Absolute  temperature=false  internal_energy=true
      settings: InternalSimscapePortConfiguration="{\"Bottom\":[{\"id\":\"U\",\"label\":\"U\",\"type\":\"output\"}],\"Left\":[{\"id\":\"A\",\"label\":\"A\",\"type\":\"foundation.two_phase_fluid.two_phase_fluid\"}],\"Right\":[{\"id\":\"B\",\"label\":\"B\",\"type\":\"foundation.two_phase_fluid.two_phase_fluid\"},{\"id\":\"P\",\"label\":\"P\",\"type\":\"output\"}],\"Top\":[]}"
  Thermodynamic Properties Sensor (2P) : fl_lib/Two-Phase Fluid/Sensors/Thermodynamic Properties Sensor (2P)  temperature=true  enthalpy=true  density=false  specific_volume=true  entropy=true
      settings: InternalSimscapePortConfiguration="{\"Bottom\":[{\"id\":\"V\",\"label\":\"v\",\"type\":\"output\"},{\"id\":\"S\",\"label\":\"s\",\"type\":\"output\"}],\"Left\":[{\"id\":\"A\",\"label\":\"A\",\"type\":\"foundation.two_phase_fluid.two_phase_fluid\"}],\"Right\":[{\"id\":\"T\",\"label\":\"T\",\"type\":\"output\"},{\"id\":\"H\",\"label\":\"h\",\"type\":\"output\"}],\"Top\":[]}"
  A : PMIOPort  Side=Left
  connections:
  Pressure & Internal Energy Sensor (2P)/LConn1 -- Thermodynamic Properties Sensor (2P)/LConn1 -- A/RConn1
  Absolute Reference (2P)/LConn1 -- Pressure & Internal Energy Sensor (2P)/RConn1

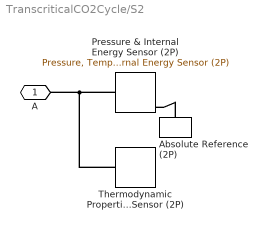
== system TranscriticalCO2Cycle/S2 ==
  Absolute Reference (2P) : fl_lib/Two-Phase Fluid/Elements/Absolute Reference (2P)
  Pressure & Internal Energy Sensor (2P) : fl_lib/Two-Phase Fluid/Sensors/Pressure, Temperature & Internal Energy Sensor (2P)  reference=foundation.enum.MeasurementReference.difference  pressure=true  pressure_spec=foundation.enum.PressureMeasementSpec.Absolute  temperature=false  internal_energy=true
      settings: InternalSimscapePortConfiguration="{\"Bottom\":[{\"id\":\"U\",\"label\":\"U\",\"type\":\"output\"}],\"Left\":[{\"id\":\"A\",\"label\":\"A\",\"type\":\"foundation.two_phase_fluid.two_phase_fluid\"}],\"Right\":[{\"id\":\"B\",\"label\":\"B\",\"type\":\"foundation.two_phase_fluid.two_phase_fluid\"},{\"id\":\"P\",\"label\":\"P\",\"type\":\"output\"}],\"Top\":[]}"
  Thermodynamic Properties Sensor (2P) : fl_lib/Two-Phase Fluid/Sensors/Thermodynamic Properties Sensor (2P)  temperature=true  enthalpy=true  density=false  specific_volume=true  entropy=true
      settings: InternalSimscapePortConfiguration="{\"Bottom\":[{\"id\":\"V\",\"label\":\"v\",\"type\":\"output\"},{\"id\":\"S\",\"label\":\"s\",\"type\":\"output\"}],\"Left\":[{\"id\":\"A\",\"label\":\"A\",\"type\":\"foundation.two_phase_fluid.two_phase_fluid\"}],\"Right\":[{\"id\":\"T\",\"label\":\"T\",\"type\":\"output\"},{\"id\":\"H\",\"label\":\"h\",\"type\":\"output\"}],\"Top\":[]}"
  A : PMIOPort  Side=Left
  connections:
  Pressure & Internal Energy Sensor (2P)/LConn1 -- Thermodynamic Properties Sensor (2P)/LConn1 -- A/RConn1
  Absolute Reference (2P)/LConn1 -- Pressure & Internal Energy Sensor (2P)/RConn1

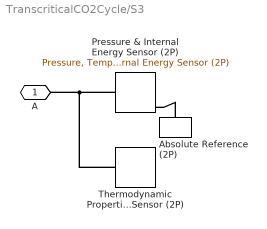
== system TranscriticalCO2Cycle/S3 ==
  Absolute Reference (2P) : fl_lib/Two-Phase Fluid/Elements/Absolute Reference (2P)
  Pressure & Internal Energy Sensor (2P) : fl_lib/Two-Phase Fluid/Sensors/Pressure, Temperature & Internal Energy Sensor (2P)  reference=foundation.enum.MeasurementReference.difference  pressure=true  pressure_spec=foundation.enum.PressureMeasementSpec.Absolute  temperature=false  internal_energy=true
      settings: InternalSimscapePortConfiguration="{\"Bottom\":[{\"id\":\"U\",\"label\":\"U\",\"type\":\"output\"}],\"Left\":[{\"id\":\"A\",\"label\":\"A\",\"type\":\"foundation.two_phase_fluid.two_phase_fluid\"}],\"Right\":[{\"id\":\"B\",\"label\":\"B\",\"type\":\"foundation.two_phase_fluid.two_phase_fluid\"},{\"id\":\"P\",\"label\":\"P\",\"type\":\"output\"}],\"Top\":[]}"
  Thermodynamic Properties Sensor (2P) : fl_lib/Two-Phase Fluid/Sensors/Thermodynamic Properties Sensor (2P)  temperature=true  enthalpy=true  density=false  specific_volume=true  entropy=true
      settings: InternalSimscapePortConfiguration="{\"Bottom\":[{\"id\":\"V\",\"label\":\"v\",\"type\":\"output\"},{\"id\":\"S\",\"label\":\"s\",\"type\":\"output\"}],\"Left\":[{\"id\":\"A\",\"label\":\"A\",\"type\":\"foundation.two_phase_fluid.two_phase_fluid\"}],\"Right\":[{\"id\":\"T\",\"label\":\"T\",\"type\":\"output\"},{\"id\":\"H\",\"label\":\"h\",\"type\":\"output\"}],\"Top\":[]}"
  A : PMIOPort  Side=Left
  connections:
  Pressure & Internal Energy Sensor (2P)/LConn1 -- Thermodynamic Properties Sensor (2P)/LConn1 -- A/RConn1
  Absolute Reference (2P)/LConn1 -- Pressure & Internal Energy Sensor (2P)/RConn1

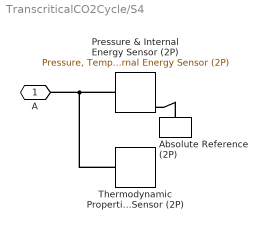
== system TranscriticalCO2Cycle/S4 ==
  Absolute Reference (2P) : fl_lib/Two-Phase Fluid/Elements/Absolute Reference (2P)
  Pressure & Internal Energy Sensor (2P) : fl_lib/Two-Phase Fluid/Sensors/Pressure, Temperature & Internal Energy Sensor (2P)  reference=foundation.enum.MeasurementReference.difference  pressure=true  pressure_spec=foundation.enum.PressureMeasementSpec.Absolute  temperature=false  internal_energy=true
      settings: InternalSimscapePortConfiguration="{\"Bottom\":[{\"id\":\"U\",\"label\":\"U\",\"type\":\"output\"}],\"Left\":[{\"id\":\"A\",\"label\":\"A\",\"type\":\"foundation.two_phase_fluid.two_phase_fluid\"}],\"Right\":[{\"id\":\"B\",\"label\":\"B\",\"type\":\"foundation.two_phase_fluid.two_phase_fluid\"},{\"id\":\"P\",\"label\":\"P\",\"type\":\"output\"}],\"Top\":[]}"
  Thermodynamic Properties Sensor (2P) : fl_lib/Two-Phase Fluid/Sensors/Thermodynamic Properties Sensor (2P)  temperature=true  enthalpy=true  density=false  specific_volume=true  entropy=true
      settings: InternalSimscapePortConfiguration="{\"Bottom\":[{\"id\":\"V\",\"label\":\"v\",\"type\":\"output\"},{\"id\":\"S\",\"label\":\"s\",\"type\":\"output\"}],\"Left\":[{\"id\":\"A\",\"label\":\"A\",\"type\":\"foundation.two_phase_fluid.two_phase_fluid\"}],\"Right\":[{\"id\":\"T\",\"label\":\"T\",\"type\":\"output\"},{\"id\":\"H\",\"label\":\"h\",\"type\":\"output\"}],\"Top\":[]}"
  A : PMIOPort  Side=Left
  connections:
  Pressure & Internal Energy Sensor (2P)/LConn1 -- Thermodynamic Properties Sensor (2P)/LConn1 -- A/RConn1
  Absolute Reference (2P)/LConn1 -- Pressure & Internal Energy Sensor (2P)/RConn1

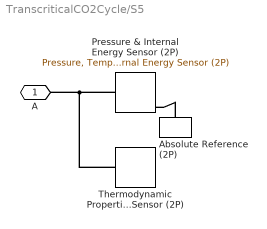
== system TranscriticalCO2Cycle/S5 ==
  Absolute Reference (2P) : fl_lib/Two-Phase Fluid/Elements/Absolute Reference (2P)
  Pressure & Internal Energy Sensor (2P) : fl_lib/Two-Phase Fluid/Sensors/Pressure, Temperature & Internal Energy Sensor (2P)  reference=foundation.enum.MeasurementReference.difference  pressure=true  pressure_spec=foundation.enum.PressureMeasementSpec.Absolute  temperature=false  internal_energy=true
      settings: InternalSimscapePortConfiguration="{\"Bottom\":[{\"id\":\"U\",\"label\":\"U\",\"type\":\"output\"}],\"Left\":[{\"id\":\"A\",\"label\":\"A\",\"type\":\"foundation.two_phase_fluid.two_phase_fluid\"}],\"Right\":[{\"id\":\"B\",\"label\":\"B\",\"type\":\"foundation.two_phase_fluid.two_phase_fluid\"},{\"id\":\"P\",\"label\":\"P\",\"type\":\"output\"}],\"Top\":[]}"
  Thermodynamic Properties Sensor (2P) : fl_lib/Two-Phase Fluid/Sensors/Thermodynamic Properties Sensor (2P)  temperature=true  enthalpy=true  density=false  specific_volume=true  entropy=true
      settings: InternalSimscapePortConfiguration="{\"Bottom\":[{\"id\":\"V\",\"label\":\"v\",\"type\":\"output\"},{\"id\":\"S\",\"label\":\"s\",\"type\":\"output\"}],\"Left\":[{\"id\":\"A\",\"label\":\"A\",\"type\":\"foundation.two_phase_fluid.two_phase_fluid\"}],\"Right\":[{\"id\":\"T\",\"label\":\"T\",\"type\":\"output\"},{\"id\":\"H\",\"label\":\"h\",\"type\":\"output\"}],\"Top\":[]}"
  A : PMIOPort  Side=Right
  connections:
  Pressure & Internal Energy Sensor (2P)/LConn1 -- Thermodynamic Properties Sensor (2P)/LConn1 -- A/RConn1
  Absolute Reference (2P)/LConn1 -- Pressure & Internal Energy Sensor (2P)/RConn1

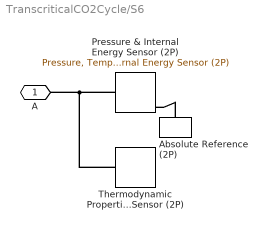
== system TranscriticalCO2Cycle/S6 ==
  Absolute Reference (2P) : fl_lib/Two-Phase Fluid/Elements/Absolute Reference (2P)
  Pressure & Internal Energy Sensor (2P) : fl_lib/Two-Phase Fluid/Sensors/Pressure, Temperature & Internal Energy Sensor (2P)  reference=foundation.enum.MeasurementReference.difference  pressure=true  pressure_spec=foundation.enum.PressureMeasementSpec.Absolute  temperature=false  internal_energy=true
      settings: InternalSimscapePortConfiguration="{\"Bottom\":[{\"id\":\"U\",\"label\":\"U\",\"type\":\"output\"}],\"Left\":[{\"id\":\"A\",\"label\":\"A\",\"type\":\"foundation.two_phase_fluid.two_phase_fluid\"}],\"Right\":[{\"id\":\"B\",\"label\":\"B\",\"type\":\"foundation.two_phase_fluid.two_phase_fluid\"},{\"id\":\"P\",\"label\":\"P\",\"type\":\"output\"}],\"Top\":[]}"
  Thermodynamic Properties Sensor (2P) : fl_lib/Two-Phase Fluid/Sensors/Thermodynamic Properties Sensor (2P)  temperature=true  enthalpy=true  density=false  specific_volume=true  entropy=true
      settings: InternalSimscapePortConfiguration="{\"Bottom\":[{\"id\":\"V\",\"label\":\"v\",\"type\":\"output\"},{\"id\":\"S\",\"label\":\"s\",\"type\":\"output\"}],\"Left\":[{\"id\":\"A\",\"label\":\"A\",\"type\":\"foundation.two_phase_fluid.two_phase_fluid\"}],\"Right\":[{\"id\":\"T\",\"label\":\"T\",\"type\":\"output\"},{\"id\":\"H\",\"label\":\"h\",\"type\":\"output\"}],\"Top\":[]}"
  A : PMIOPort  Side=Left
  connections:
  Pressure & Internal Energy Sensor (2P)/LConn1 -- Thermodynamic Properties Sensor (2P)/LConn1 -- A/RConn1
  Absolute Reference (2P)/LConn1 -- Pressure & Internal Energy Sensor (2P)/RConn1

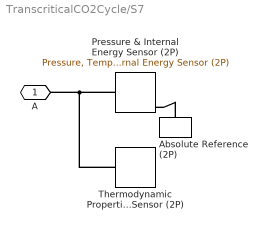
== system TranscriticalCO2Cycle/S7 ==
  Absolute Reference (2P) : fl_lib/Two-Phase Fluid/Elements/Absolute Reference (2P)
  Pressure & Internal Energy Sensor (2P) : fl_lib/Two-Phase Fluid/Sensors/Pressure, Temperature & Internal Energy Sensor (2P)  reference=foundation.enum.MeasurementReference.difference  pressure=true  pressure_spec=foundation.enum.PressureMeasementSpec.Absolute  temperature=false  internal_energy=true
      settings: InternalSimscapePortConfiguration="{\"Bottom\":[{\"id\":\"U\",\"label\":\"U\",\"type\":\"output\"}],\"Left\":[{\"id\":\"A\",\"label\":\"A\",\"type\":\"foundation.two_phase_fluid.two_phase_fluid\"}],\"Right\":[{\"id\":\"B\",\"label\":\"B\",\"type\":\"foundation.two_phase_fluid.two_phase_fluid\"},{\"id\":\"P\",\"label\":\"P\",\"type\":\"output\"}],\"Top\":[]}"
  Thermodynamic Properties Sensor (2P) : fl_lib/Two-Phase Fluid/Sensors/Thermodynamic Properties Sensor (2P)  temperature=true  enthalpy=true  density=false  specific_volume=true  entropy=true
      settings: InternalSimscapePortConfiguration="{\"Bottom\":[{\"id\":\"V\",\"label\":\"v\",\"type\":\"output\"},{\"id\":\"S\",\"label\":\"s\",\"type\":\"output\"}],\"Left\":[{\"id\":\"A\",\"label\":\"A\",\"type\":\"foundation.two_phase_fluid.two_phase_fluid\"}],\"Right\":[{\"id\":\"T\",\"label\":\"T\",\"type\":\"output\"},{\"id\":\"H\",\"label\":\"h\",\"type\":\"output\"}],\"Top\":[]}"
  A : PMIOPort  Side=Left
  connections:
  Pressure & Internal Energy Sensor (2P)/LConn1 -- Thermodynamic Properties Sensor (2P)/LConn1 -- A/RConn1
  Absolute Reference (2P)/LConn1 -- Pressure & Internal Energy Sensor (2P)/RConn1

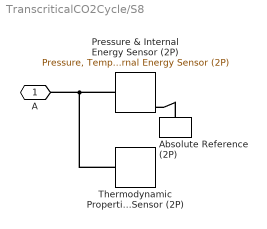
== system TranscriticalCO2Cycle/S8 ==
  Absolute Reference (2P) : fl_lib/Two-Phase Fluid/Elements/Absolute Reference (2P)
  Pressure & Internal Energy Sensor (2P) : fl_lib/Two-Phase Fluid/Sensors/Pressure, Temperature & Internal Energy Sensor (2P)  reference=foundation.enum.MeasurementReference.difference  pressure=true  pressure_spec=foundation.enum.PressureMeasementSpec.Absolute  temperature=false  internal_energy=true
      settings: InternalSimscapePortConfiguration="{\"Bottom\":[{\"id\":\"U\",\"label\":\"U\",\"type\":\"output\"}],\"Left\":[{\"id\":\"A\",\"label\":\"A\",\"type\":\"foundation.two_phase_fluid.two_phase_fluid\"}],\"Right\":[{\"id\":\"B\",\"label\":\"B\",\"type\":\"foundation.two_phase_fluid.two_phase_fluid\"},{\"id\":\"P\",\"label\":\"P\",\"type\":\"output\"}],\"Top\":[]}"
  Thermodynamic Properties Sensor (2P) : fl_lib/Two-Phase Fluid/Sensors/Thermodynamic Properties Sensor (2P)  temperature=true  enthalpy=true  density=false  specific_volume=true  entropy=true
      settings: InternalSimscapePortConfiguration="{\"Bottom\":[{\"id\":\"V\",\"label\":\"v\",\"type\":\"output\"},{\"id\":\"S\",\"label\":\"s\",\"type\":\"output\"}],\"Left\":[{\"id\":\"A\",\"label\":\"A\",\"type\":\"foundation.two_phase_fluid.two_phase_fluid\"}],\"Right\":[{\"id\":\"T\",\"label\":\"T\",\"type\":\"output\"},{\"id\":\"H\",\"label\":\"h\",\"type\":\"output\"}],\"Top\":[]}"
  A : PMIOPort  Side=Right
  connections:
  Pressure & Internal Energy Sensor (2P)/LConn1 -- Thermodynamic Properties Sensor (2P)/LConn1 -- A/RConn1
  Absolute Reference (2P)/LConn1 -- Pressure & Internal Energy Sensor (2P)/RConn1
